simulink model "PMSM_Simulink"  (R2024b)
settings: Solver=FixedStepDiscrete  StartTime=0.0  StopTime=10  FixedStep=0.0000625/200  RelTol=1e-3
libraries: simulink x12, slpidlib x3, spsDCVoltageSourceLib x1, spsPermanentMagnetSynchronousMachineLib x1, spsUniversalBridgeLib x1, sps_lib x1
(part 1 of 2)
settings Model: SimulationMode=accelerator  PacingRate=1000  Creator=1111  LastModifiedBy=1111
settings OptimizationCC: DefaultParameterBehavior=Inlined  EnhancedBackFolding=on  PassReuseOutputArgsAs=Individual arguments  ZeroExternalMemoryAtStartup=off  ZeroInternalMemoryAtStartup=off  OptimizeBlockOrder=speed  DifferentSizesBufferReuse=on  OptimizationCustomize=off  EfficientTunableParamExpr=on
settings DebuggingCC: ParameterPrecisionLossMsg=none  ParameterTunabilityLossMsg=error
settings SFSimCC: MATLABDynamicMemAlloc=off
settings RTWCC: Description=Embedded Coder  SystemTargetFile=ert.tlc  TemplateMakefile=ert_default_tmf
settings CodeAppCC: ForceParamTrailComments=on  IgnoreCustomStorageClasses=off  OperatorAnnotations=on  SimulinkDataObjDesc=on  SFDataObjDesc=on  InsertBlockDesc=on
settings ERTTargetCC: TargetLangStandard=C99 (ISO)  GenerateSampleERTMain=on  ERTCustomFileTemplate=example_file_process.tlc

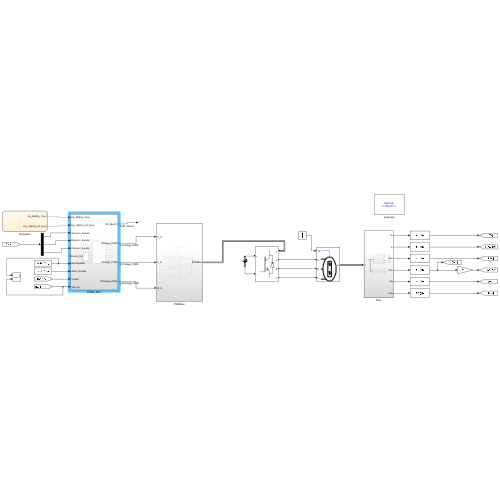
[thumbnail: Simulink's stored preview of the top-level diagram]
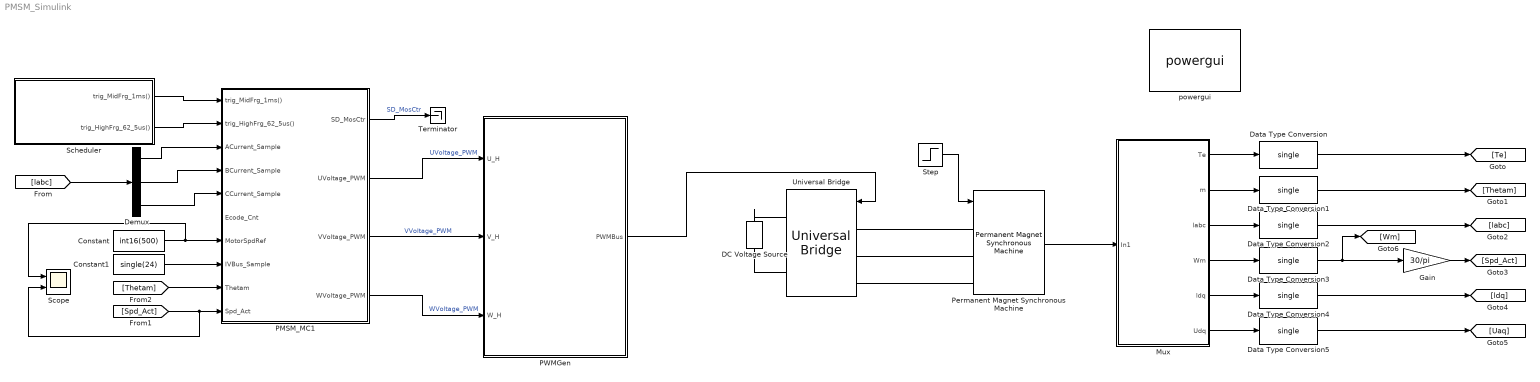
== system PMSM_Simulink ==
  Constant : Constant  Value=int16(500)  OutDataTypeStr=int16
  Constant1 : Constant  Value=single(24)
  DC Voltage Source : spsDCVoltageSourceLib/DC Voltage Source  Amplitude=24  Measurements=None
  Data Type Conversion{,1..5} (6 alike) : DataTypeConversion  OutDataTypeStr=single  SaturateOnIntegerOverflow=off  RndMeth=Floor
  Demux : Demux  Outputs=3
  Gain : Gain  Gain=30/pi
  Mux : Subsystem
  PMSM_MC1 : Subsystem
  PWMGen : Subsystem
  Permanent Magnet Synchronous Machine : spsPermanentMagnetSynchronousMachineLib/Permanent Magnet Synchronous Machine  NbPhases=3  FluxDistribution=Sinusoidal  RotorType=Salient-pole  MechanicalLoad=Torque Tm  PresetModel=No  ShowDetailedParameters=on  MeasurementBus=off  Resistance=0.51  Inductance=8.5e-3  dqInductances=[0.295e-3,0.295e-3]  La=0.00086  MachineConstant=Flux linkage established by magnets (V.s)  Flux=0.00838  VoltageCst=6.0799  TorqueCst=0.05028  Flat=120  Mechanical=[0.0000028 0 4 0 ]  PolePairs=4  InitialConditions=[0,0, 0,0]  InitialConditions5ph=[0 0 0 0 0 0]  RefAngle=Aligned with phase A axis (original Park)  IterativeDiscreteModel=Trapezoidal non iterative  TsBlock=-1  TsPowergui=0
  Scheduler : Stateflow chart  TreatAsAtomicUnit=on
  Scope : Scope  NumInputPorts=2
  Step : Step  Time=0  After=0  SampleTime=0
  Terminator : Terminator
  Universal Bridge : spsUniversalBridgeLib/Universal Bridge  Arms=3  SnubberResistance=1e5  SnubberCapacitance=inf  Device=IGBT / Diodes  Ron=1e-3  Lon=0  ForwardVoltages="[  0  0  ]"  ForwardVoltage=0  GTOparameters=[ 10e-6 , 20e-6 ]  IGBTparameters=[ 1e-6 , 2e-6 ]  Measurements=None  Measurements_2=None  converterType=Rectifier
  powergui : sps_lib/powergui  Priority=1  SimulationMode=Discrete  SampleTime=0.0000625/200  frequency=60  Iterations=50  frequencyindice=0  Pbase=100e6  ErrMax=1e-4  UnitsV=kV  UnitsW=MW  buscounter=0  FunctionMessages=off  echomessages=off  EnableUseOfTLC=off  CurrentSourceSwitches=off  DisableSnubberDevices=off  DisableRonSwitches=off  DisableVfSwitches=off  DisplayEquations=off  AutomaticDiscreteSolvers=off  SolverType=Tustin/Backward Euler (TBE)  Interpol=off  ExternalGateDelay=off  methode=off  Ts=100  x0status=blocks  SPID=on  SwTol=0  HookPort=off  NonlinearTolerance=1e-4  nMaxIteration=100  ContinueOnMaxIteration=off  RestoreLinks=warning  ResistiveCurrentMeasurement=off  Frange=[0:2:500]  Ylog=off  Xlog=on  ShowGrid=off  save=off  variable=ZData  structure=0  ZoomFFT=off  StartTime=0.0  cycles=1  DisplayStyle=1  fundamental=60  FreqAxis=off  MaxFrequency=1000  frequencyindicesteady=1  RmsSteady=1  display=off
  wires:
  Step/1 -> Permanent Magnet Synchronous Machine/1
  PWMGen/1(PWMBus) -> Universal Bridge/1
  Permanent Magnet Synchronous Machine/1 -> Mux/1(In1)
  Mux/1(Te) -> Data Type Conversion/1
  Mux/2(m) -> Data Type Conversion1/1
  Mux/3(labc) -> Data Type Conversion2/1
  Mux/4(Wm) -> Data Type Conversion3/1
  Mux/5(ldq) -> Data Type Conversion4/1
  Mux/6(Udq) -> Data Type Conversion5/1
  Data Type Conversion3/1 -> [Wm], Gain/1
  Data Type Conversion/1 -> [Te]
  Data Type Conversion1/1 -> [Thetam]
  Data Type Conversion2/1 -> [labc]
  Gain/1 -> [Spd_Act]
  Data Type Conversion4/1 -> [ldq]
  Data Type Conversion5/1 -> [Uaq]
  [labc] -> Demux/1
  PMSM_MC1/1(SD_MosCtr) -> Terminator/1  "SD_MosCtr"
  PMSM_MC1/3(VVoltage_PWM) -> PWMGen/2(V_H)  "VVoltage_PWM"
  PMSM_MC1/2(UVoltage_PWM) -> PWMGen/1(U_H)  "UVoltage_PWM"
  PMSM_MC1/4(WVoltage_PWM) -> PWMGen/3(W_H)  "WVoltage_PWM"
  Scheduler/1(trig_MidFrg_1ms()) -> PMSM_MC1/1(trig_MidFrg_1ms())
  Scheduler/2(trig_HighFrg_62_5us()) -> PMSM_MC1/2(trig_HighFrg_62_5us())
  Demux/1 -> PMSM_MC1/3(ACurrent_Sample)
  Demux/2 -> PMSM_MC1/4(BCurrent_Sample)
  Demux/3 -> PMSM_MC1/5(CCurrent_Sample)
  Constant/1 -> Scope/1, PMSM_MC1/7(MotorSpdRef)
  Constant1/1 -> PMSM_MC1/8(IVBus_Sample)
  [Thetam] -> PMSM_MC1/9(Thetam)
  [Spd_Act] -> Scope/2, PMSM_MC1/10(Spd_Act)
  connections:
  DC Voltage Source/LConn1 -- Universal Bridge/RConn2
  DC Voltage Source/RConn1 -- Universal Bridge/RConn1
  Universal Bridge/LConn2 -- Permanent Magnet Synchronous Machine/LConn2
  Universal Bridge/LConn1 -- Permanent Magnet Synchronous Machine/LConn1
  Universal Bridge/LConn3 -- Permanent Magnet Synchronous Machine/LConn3

== system PMSM_Simulink/Mux ==
  In1 : Inport
  Bus Selector : BusSelector  OutputSignals=Stator current is_a (A),Stator current is_b (A),Stator current is_c (A),Stator current is_q (A),Stator current is_d (A),Stator voltage Vs_q (V),Stator voltage Vs_d (V)
  Bus Selector1 : BusSelector  OutputSignals=Rotor speed wm (rad/s),Rotor angle thetam (rad),Electromagnetic torque Te (N*m)
  Mux : Mux  Inputs=3
  Mux1 : Mux  Inputs=2
  Mux2 : Mux  Inputs=2
  Te : Outport
  m : Outport  Port=2
  labc : Outport  Port=3
  Wm : Outport  Port=4
  ldq : Outport  Port=5
  Udq : Outport  Port=6
  wires:
  In1/1 -> Bus Selector1/1, Bus Selector/1
  Mux/1 -> labc/1
  Mux1/1 -> ldq/1
  Mux2/1 -> Udq/1
  Bus Selector/1 -> Mux/1  "<Stator current is_a (A)>"
  Bus Selector/2 -> Mux/2  "<Stator current is_b (A)>"
  Bus Selector/3 -> Mux/3  "<Stator current is_c (A)>"
  Bus Selector/4 -> Mux1/1  "<Stator current is_q (A)>"
  Bus Selector/5 -> Mux1/2  "<Stator current is_d (A)>"
  Bus Selector/6 -> Mux2/1  "<Stator voltage Vs_q (V)>"
  Bus Selector/7 -> Mux2/2  "<Stator voltage Vs_d (V)>"
  Bus Selector1/1 -> Wm/1  "<Rotor speed wm (rad/s)>"
  Bus Selector1/2 -> m/1  "<Rotor angle thetam (rad)>"
  Bus Selector1/3 -> Te/1  "<Electromagnetic torque Te (N*m)>"

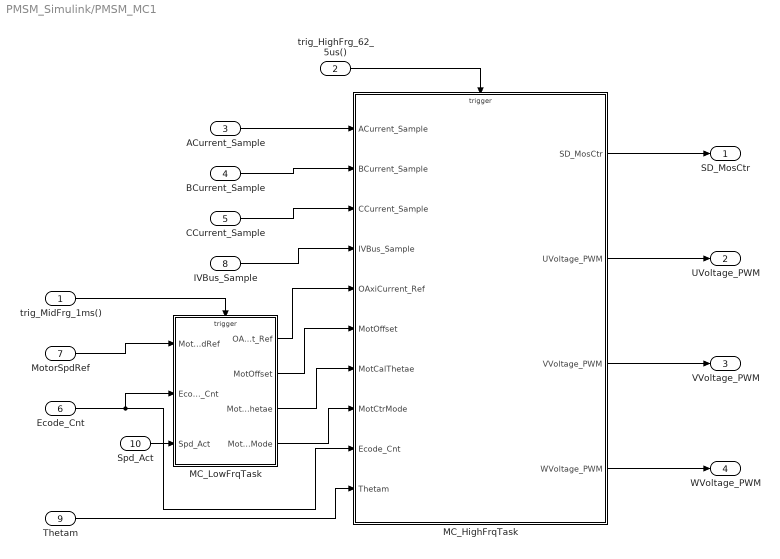
== system PMSM_Simulink/PMSM_MC1 ==
  trig_MidFrg_1ms() : Inport
  trig_HighFrg_62_5us() : Inport  Port=2
  ACurrent_Sample : Inport  Port=3
  BCurrent_Sample : Inport  Port=4
  CCurrent_Sample : Inport  Port=5
  Ecode_Cnt : Inport  Port=6
  MotorSpdRef : Inport  Port=7  OutDataTypeStr=int16
  IVBus_Sample : Inport  Port=8
  Thetam : Inport  Port=9
  Spd_Act : Inport  Port=10
  MC_HighFrqTask : Subsystem  TreatAsAtomicUnit=on
  "MC_LowFrqTask " : Subsystem  TreatAsAtomicUnit=on
  SD_MosCtr : Outport
  UVoltage_PWM : Outport  Port=2
  VVoltage_PWM : Outport  Port=3
  WVoltage_PWM : Outport  Port=4
  wires:
  trig_MidFrg_1ms()/1 -> "MC_LowFrqTask "/Trigger
  trig_HighFrg_62_5us()/1 -> MC_HighFrqTask/Trigger
  MotorSpdRef/1 -> "MC_LowFrqTask "/1(MotorSpdRef)
  Ecode_Cnt/1 -> MC_HighFrqTask/9(Ecode_Cnt), "MC_LowFrqTask "/2(Ecode_Cnt)
  ACurrent_Sample/1 -> MC_HighFrqTask/1(ACurrent_Sample)
  BCurrent_Sample/1 -> MC_HighFrqTask/2(BCurrent_Sample)
  CCurrent_Sample/1 -> MC_HighFrqTask/3(CCurrent_Sample)
  IVBus_Sample/1 -> MC_HighFrqTask/4(IVBus_Sample)
  "MC_LowFrqTask "/4(MotCtrMode) -> MC_HighFrqTask/8(MotCtrMode)
  "MC_LowFrqTask "/3(MotCalThetae) -> MC_HighFrqTask/7(MotCalThetae)
  "MC_LowFrqTask "/2(MotOffset) -> MC_HighFrqTask/6(MotOffset)
  "MC_LowFrqTask "/1(OAxiCurrent_Ref) -> MC_HighFrqTask/5(OAxiCurrent_Ref)
  MC_HighFrqTask/1(SD_MosCtr) -> SD_MosCtr/1
  MC_HighFrqTask/2(UVoltage_PWM) -> UVoltage_PWM/1
  MC_HighFrqTask/3(VVoltage_PWM) -> VVoltage_PWM/1
  MC_HighFrqTask/4(WVoltage_PWM) -> WVoltage_PWM/1
  Spd_Act/1 -> "MC_LowFrqTask "/3(Spd_Act)
  Thetam/1 -> MC_HighFrqTask/10(Thetam)

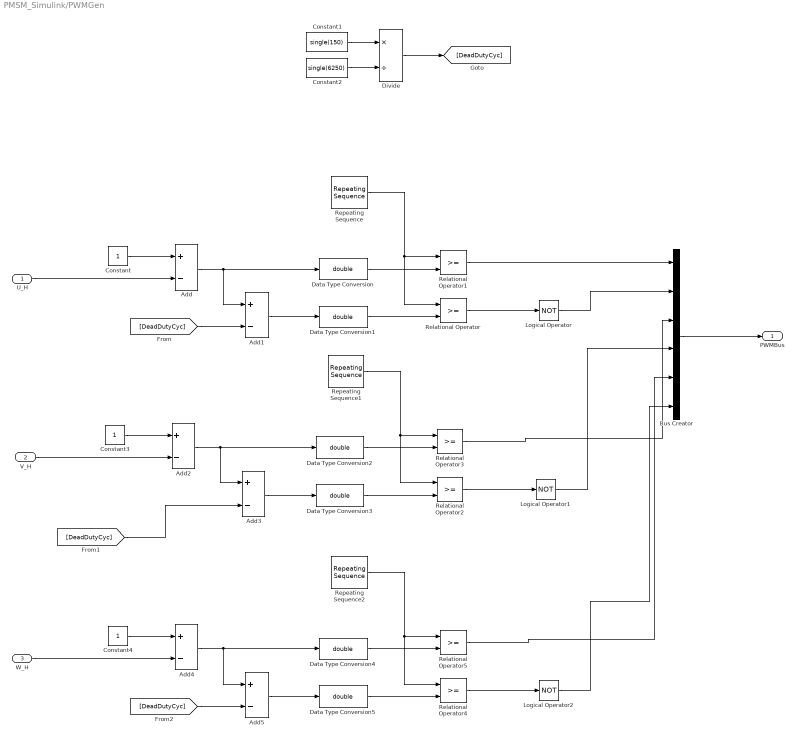
== system PMSM_Simulink/PWMGen ==
  U_H : Inport
  V_H : Inport  Port=2
  W_H : Inport  Port=3
  Add{,1..5} (6 alike) : Sum  Inputs=+-
  Bus Creator : BusCreator  Inputs=6
  Constant : Constant
  Constant1 : Constant  Value=single(150)
  Constant2 : Constant  Value=single(6250)
  Constant3 : Constant
  Constant4 : Constant
  Data Type Conversion{,1..5} (6 alike) : DataTypeConversion  OutDataTypeStr=double  SaturateOnIntegerOverflow=off  RndMeth=Floor
  Divide : Product  Inputs=*/
  Logical Operator : Logic  Operator=NOT  AllPortsSameDT=off  OutDataTypeStr=boolean
  Logical Operator1 : Logic  Operator=NOT  AllPortsSameDT=off  OutDataTypeStr=boolean
  Logical Operator2 : Logic  Operator=NOT  AllPortsSameDT=off  OutDataTypeStr=boolean
  Relational Operator{,1..5} (6 alike) : RelationalOperator  OutDataTypeStr=boolean  RndMeth=Simplest  InputSameDT=off
  Repeating Sequence : simulink/Sources/Repeating Sequence  rep_seq_t=[0 0.0000625/2 0.0000625]  rep_seq_y=[0 1 0]
  Repeating Sequence1 : simulink/Sources/Repeating Sequence  rep_seq_t=[0 0.0000625/2 0.0000625]  rep_seq_y=[0 1 0]
  Repeating Sequence2 : simulink/Sources/Repeating Sequence  rep_seq_t=[0 0.0000625/2 0.0000625]  rep_seq_y=[0 1 0]
  PWMBus : Outport
  wires:
  U_H/1 -> Add/2
  Constant/1 -> Add/1
  Add/1 -> Data Type Conversion/1, Add1/1
  Add1/1 -> Data Type Conversion1/1
  Data Type Conversion1/1 -> Relational Operator/2
  Data Type Conversion/1 -> Relational Operator1/2
  Repeating Sequence/1 -> Relational Operator/1, Relational Operator1/1
  Relational Operator/1 -> Logical Operator/1
  Relational Operator1/1 -> Bus Creator/1
  Logical Operator/1 -> Bus Creator/2
  Constant1/1 -> Divide/1
  Constant2/1 -> Divide/2
  Divide/1 -> [DeadDutyCyc]
  [DeadDutyCyc] -> Add1/2
  [DeadDutyCyc] -> Add3/2
  Relational Operator2/1 -> Logical Operator1/1
  Data Type Conversion2/1 -> Relational Operator3/2
  Data Type Conversion3/1 -> Relational Operator2/2
  Constant3/1 -> Add2/1
  Repeating Sequence1/1 -> Relational Operator2/1, Relational Operator3/1
  Add2/1 -> Data Type Conversion2/1, Add3/1
  Logical Operator1/1 -> Bus Creator/4
  V_H/1 -> Add2/2
  Add3/1 -> Data Type Conversion3/1
  Relational Operator3/1 -> Bus Creator/3
  [DeadDutyCyc] -> Add5/2
  Relational Operator4/1 -> Logical Operator2/1
  Data Type Conversion4/1 -> Relational Operator5/2
  Data Type Conversion5/1 -> Relational Operator4/2
  Constant4/1 -> Add4/1
  Repeating Sequence2/1 -> Relational Operator4/1, Relational Operator5/1
  Add4/1 -> Data Type Conversion4/1, Add5/1
  Logical Operator2/1 -> Bus Creator/6
  W_H/1 -> Add4/2
  Add5/1 -> Data Type Conversion5/1
  Relational Operator5/1 -> Bus Creator/5
  Bus Creator/1 -> PWMBus/1

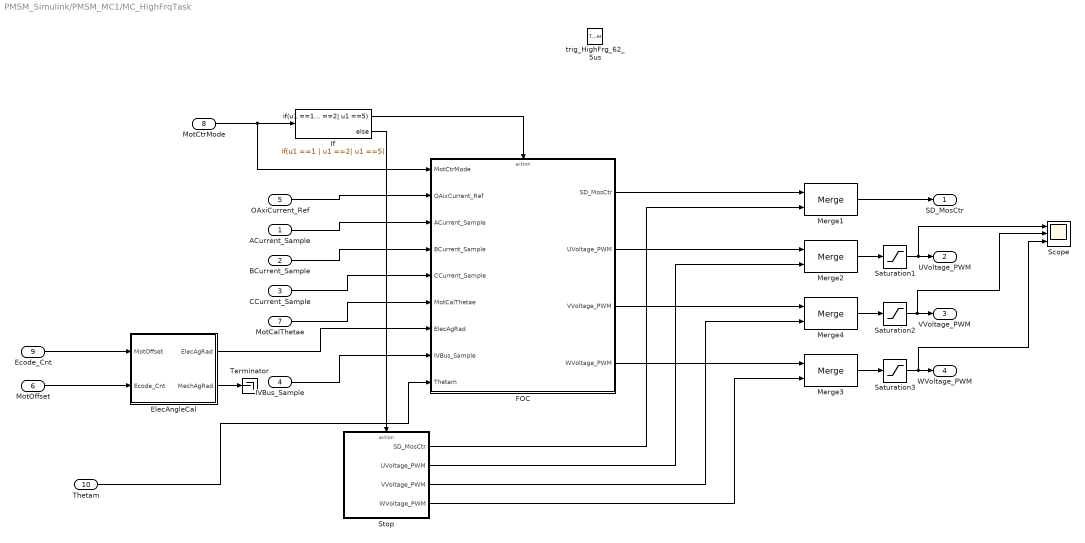
== system PMSM_Simulink/PMSM_MC1/MC_HighFrqTask ==
  ACurrent_Sample : Inport
  BCurrent_Sample : Inport  Port=2
  CCurrent_Sample : Inport  Port=3
  IVBus_Sample : Inport  Port=4
  OAxiCurrent_Ref : Inport  Port=5
  MotOffset : Inport  Port=6
  MotCalThetae : Inport  Port=7
  MotCtrMode : Inport  Port=8
  Ecode_Cnt : Inport  Port=9
  Thetam : Inport  Port=10
  trig_HighFrg_62_5us : TriggerPort  TriggerType=function-call  VariantControl=(inherit)
  ElecAngleCal : Subsystem
  FOC : Subsystem  TreatAsAtomicUnit=on
  If : If  IfExpression=u1 ==1 | u1 ==2| u1 ==5
  Merge{1..4} (4 alike) : Merge
  Saturation1 : Saturate  UpperLimit=0.95  LowerLimit=0
  Saturation2 : Saturate  UpperLimit=0.95  LowerLimit=0
  Saturation3 : Saturate  UpperLimit=0.95  LowerLimit=0
  Scope : Scope  NumInputPorts=3
  Stop : Subsystem  TreatAsAtomicUnit=on
  Terminator : Terminator
  SD_MosCtr : Outport
  UVoltage_PWM : Outport  Port=2
  VVoltage_PWM : Outport  Port=3
  WVoltage_PWM : Outport  Port=4
  wires:
  MotCtrMode/1 -> FOC/1(MotCtrMode), If/1
  If/1 -> FOC/Action
  If/2 -> Stop/Action
  FOC/1(SD_MosCtr) -> Merge1/1
  FOC/2(UVoltage_PWM) -> Merge2/1
  FOC/3(VVoltage_PWM) -> Merge4/1
  FOC/4(WVoltage_PWM) -> Merge3/1
  Stop/1(SD_MosCtr) -> Merge1/2
  Stop/2(UVoltage_PWM) -> Merge2/2
  Stop/3(VVoltage_PWM) -> Merge4/2
  Stop/4(WVoltage_PWM) -> Merge3/2
  Merge2/1 -> Saturation1/1
  Merge4/1 -> Saturation2/1
  Merge3/1 -> Saturation3/1
  Saturation1/1 -> Scope/1, UVoltage_PWM/1
  Saturation2/1 -> Scope/2, VVoltage_PWM/1
  Saturation3/1 -> Scope/3, WVoltage_PWM/1
  Merge1/1 -> SD_MosCtr/1
  Ecode_Cnt/1 -> ElecAngleCal/1(MotOffset)
  MotOffset/1 -> ElecAngleCal/2(Ecode_Cnt)
  ACurrent_Sample/1 -> FOC/3(ACurrent_Sample)
  BCurrent_Sample/1 -> FOC/4(BCurrent_Sample)
  CCurrent_Sample/1 -> FOC/5(CCurrent_Sample)
  OAxiCurrent_Ref/1 -> FOC/2(QAixCurrent_Ref)
  MotCalThetae/1 -> FOC/6(MotCalThetae)
  IVBus_Sample/1 -> FOC/8(IVBus_Sample)
  ElecAngleCal/1(ElecAgRad) -> FOC/7(ElecAgRad)
  ElecAngleCal/2(MechAgRad) -> Terminator/1
  Thetam/1 -> FOC/9(Thetam)

== system PMSM_Simulink/PMSM_MC1/MC_LowFrqTask  ==
  MotorSpdRef : Inport  OutDataTypeStr=int16
  Ecode_Cnt : Inport  Port=2
  Spd_Act : Inport  Port=3
  trig_MidFrg_1ms : TriggerPort  TriggerType=function-call  VariantControl=(inherit)
  MotModeCtr : Subsystem
  MotSpdCal : Subsystem
  SpdLoop : Subsystem
  OAxiCurrent_Ref : Outport
  MotOffset : Outport  Port=2
  MotCalThetae : Outport  Port=3
  MotCtrMode : Outport  Port=4  OutDataTypeStr=single
  wires:
  MotorSpdRef/1 -> SpdLoop/2(MotorSpdRef), MotModeCtr/2(MotorSpdRef)
  SpdLoop/1(OAxiCurrent_Ref) -> OAxiCurrent_Ref/1
  Spd_Act/1 -> SpdLoop/3(MotorActSpd)
  MotModeCtr/1(MotOffset) -> MotOffset/1
  MotModeCtr/2(MotCalThetae) -> MotCalThetae/1
  MotModeCtr/3(MotCtrMode) -> SpdLoop/1(MotorSpdRef1), MotCtrMode/1
  Ecode_Cnt/1 -> MotSpdCal/1(Ecode_Cnt), MotModeCtr/1(Ecdoe_Crt)

== system PMSM_Simulink/PMSM_MC1/MC_HighFrqTask/ElecAngleCal ==
  MotOffset : Inport
  Ecode_Cnt : Inport  Port=2
  Add : Sum  Inputs=+-
  AngleCal : Subsystem
  Demux : Demux  Outputs=2
  ElecAgRad : Outport
  MechAgRad : Outport  Port=2
  wires:
  Ecode_Cnt/1 -> Add/1
  MotOffset/1 -> Add/2
  Add/1 -> AngleCal/1(Ecode_CntCorrect)
  AngleCal/1(Theat) -> Demux/1
  Demux/2 -> ElecAgRad/1
  Demux/1 -> MechAgRad/1

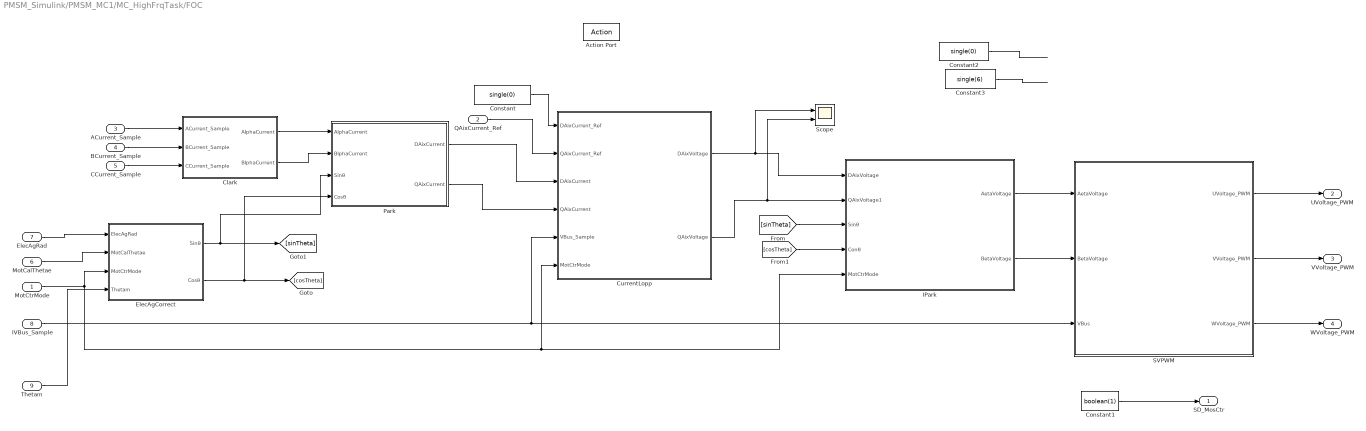
== system PMSM_Simulink/PMSM_MC1/MC_HighFrqTask/FOC ==
  MotCtrMode : Inport
  QAixCurrent_Ref : Inport  Port=2
  ACurrent_Sample : Inport  Port=3
  BCurrent_Sample : Inport  Port=4
  CCurrent_Sample : Inport  Port=5
  MotCalThetae : Inport  Port=6
  ElecAgRad : Inport  Port=7
  IVBus_Sample : Inport  Port=8
  Thetam : Inport  Port=9
  Action Port : ActionPort  ActionPortLabel=if(u1 ==1 | u1 ==2| u1 ==5)
  Clark : Subsystem
  Constant : Constant  Value=single(0)
  Constant1 : Constant  Value=boolean(1)
  Constant2 : Constant  Value=single(0)
  Constant3 : Constant  Value=single(6)
  CurrentLopp : Subsystem
  ElecAgCorrect : Subsystem
  IPark : Subsystem
  Park : Subsystem
  SVPWM : Subsystem
  Scope : Scope  NumInputPorts=2
  SD_MosCtr : Outport
  UVoltage_PWM : Outport  Port=2
  VVoltage_PWM : Outport  Port=3
  WVoltage_PWM : Outport  Port=4
  wires:
  Park/2(QAixCurrent) -> CurrentLopp/4(QAixCurrent)
  Clark/2(BIphaCurrent) -> Park/2(BIphaCurrent)
  Park/1(DAixCurrent) -> CurrentLopp/3(DAixCurrent)
  IPark/1(AetaVoltage) -> SVPWM/1(AetaVoltage)
  IPark/2(BetaVoltage) -> SVPWM/2(BetaVoltage)
  QAixCurrent_Ref/1 -> CurrentLopp/2(QAixCurrent_Ref)
  Constant/1 -> CurrentLopp/1(DAixCurrent_Ref)
  Clark/1(AIphaCurrent) -> Park/1(AIphaCurrent)
  ACurrent_Sample/1 -> Clark/1(ACurrent_Sample)
  CCurrent_Sample/1 -> Clark/3(CCurrent_Sample)
  BCurrent_Sample/1 -> Clark/2(BCurrent_Sample)
  ElecAgRad/1 -> ElecAgCorrect/1(ElecAgRad)
  MotCalThetae/1 -> ElecAgCorrect/2(MotCalThetae)
  MotCtrMode/1 -> CurrentLopp/6(MotCtrMode), IPark/5(MotCtrMode), ElecAgCorrect/3(MotCtrMode)
  ElecAgCorrect/1(Sinθ) -> Park/3(Sinθ), [sinTheta]
  ElecAgCorrect/2(Cosθ) -> Park/4(Cosθ), [cosTheta]
  [sinTheta] -> IPark/3(Sinθ)
  [cosTheta] -> IPark/4(Conθ)
  IVBus_Sample/1 -> CurrentLopp/5(VBus_Sample), SVPWM/3(VBus)
  SVPWM/2(VVoltage_PWM) -> VVoltage_PWM/1
  SVPWM/1(UVoltage_PWM) -> UVoltage_PWM/1
  SVPWM/3(WVoltage_PWM) -> WVoltage_PWM/1
  Constant1/1 -> SD_MosCtr/1
  Thetam/1 -> ElecAgCorrect/4(Thetam)
  Constant2/1 -> ?
  Constant3/1 -> ?
  CurrentLopp/2(QAixVoltage) -> Scope/2, IPark/2(QAixVoltage1)
  CurrentLopp/1(DAixVoltage) -> Scope/1, IPark/1(DAixVoltage)

== system PMSM_Simulink/PMSM_MC1/MC_HighFrqTask/Stop ==
  Action Port : ActionPort  ActionPortLabel=else
  Constant : Constant  Value=single(0)
  Constant1 : Constant  Value=boolean(0)
  SD_MosCtr : Outport
  UVoltage_PWM : Outport  Port=2
  VVoltage_PWM : Outport  Port=3
  WVoltage_PWM : Outport  Port=4
  wires:
  Constant/1 -> WVoltage_PWM/1, VVoltage_PWM/1, UVoltage_PWM/1
  Constant1/1 -> SD_MosCtr/1

== system PMSM_Simulink/PMSM_MC1/MC_LowFrqTask /MotModeCtr ==
  Ecdoe_Crt : Inport
  MotorSpdRef : Inport  Port=2  OutDataTypeStr=int16
  Chart : Stateflow chart  TreatAsAtomicUnit=on
  Compare To Constant : simulink/Logic and Bit Operations/Compare To Constant  relop=~=  const=255  OutDataTypeStr=boolean
  Constant : Constant  Value=5  OutDataTypeStr=uint8
  Switch : Switch  Criteria=u2 > Threshold  OutDataTypeStr=single  SaturateOnIntegerOverflow=off  InputSameDT=off
  MotOffset : Outport
  MotCalThetae : Outport  Port=2
  MotCtrMode : Outport  Port=3
  wires:
  Chart/2(MotOffset) -> MotOffset/1
  Chart/3(MotCalThetae) -> MotCalThetae/1
  MotorSpdRef/1 -> Chart/1(MotorSpdRef)
  Ecdoe_Crt/1 -> Chart/2(Ecode_Cnt)
  Switch/1 -> MotCtrMode/1
  Chart/1(MotCtrMode) -> Switch/3
  Compare To Constant/1 -> Switch/2
  Constant/1 -> Switch/1, Compare To Constant/1

== system PMSM_Simulink/PMSM_MC1/MC_LowFrqTask /MotSpdCal ==
  Ecode_Cnt : Inport
  Constant : Constant  Value=single(4000)
  Constant1 : Constant  Value=single(60000)
  Constant2 : Constant  Value=single(1)
  Data Type Conversion : DataTypeConversion  OutDataTypeStr=single  SaturateOnIntegerOverflow=off  RndMeth=Floor
  Delay : Delay  DelayLength=1  InitialConditionSource=Input port
      settings: InputPortMap=u0,p4
  Divide : Product  Inputs=*/
  Minus : Sum  Inputs=+-
  Product : Product
  Subsystem : Subsystem
  MotorActSpd : Outport
  wires:
  Delay/1 -> Minus/2
  Ecode_Cnt/1 -> Delay/2, Delay/1, Minus/1
  Data Type Conversion/1 -> Divide/1
  Minus/1 -> Data Type Conversion/1
  Constant/1 -> Divide/2
  Constant1/1 -> Product/2
  Divide/1 -> Product/1
  Product/1 -> Subsystem/1(In)
  Subsystem/1(MotorActSpd) -> MotorActSpd/1
  Constant2/1 -> Subsystem/2(TiCon)

== system PMSM_Simulink/PMSM_MC1/MC_LowFrqTask /SpdLoop ==
  MotorSpdRef1 : Inport
  MotorSpdRef : Inport  Port=2
  MotorActSpd : Inport  Port=3
  Compare To Constant : simulink/Logic and Bit Operations/Compare To Constant  relop===  const=5  OutDataTypeStr=boolean
  Constant1 : Constant  Value=single(6)
  Constant2 : Constant  Value=0  OutDataTypeStr=single
  Constant3 : Constant  Value=0.0001  OutDataTypeStr=single
  Constant4 : Constant  Value=0.006  OutDataTypeStr=single
  Data Type Conversion : DataTypeConversion  OutDataTypeStr=single  SaturateOnIntegerOverflow=off  RndMeth=Floor
  Discrete PID Controller : slpidlib/PID Controller  Controller=PI  Form=Parallel  TimeDomain=Discrete-time  UseExternalTs=off  SampleTime=-1  IntegratorMethod=Forward Euler  FilterMethod=Forward Euler  ControllerParametersSource=external  P=1  I=1  UseKiTs=on  D=0  UseExternalDerivativeSource=off  N=100  UseFilter=on  TunerSelectOption=Transfer Function Based (PID Tuner App)  InitialConditionSource=external  InitialConditionForIntegrator=0  InitialConditionForFilter=0  DifferentiatorICPrevScaledInput=0  ExternalReset=rising  TrackingMode=off  Kt=1  LimitOutput=off  SatLimitsSource=external  UpperSaturationLimit=inf  LowerSaturationLimit=-inf  LinearizeAsGain=off  AntiWindupMode=none  Kb=1  LimitIntegrator=on  UpperIntegratorSaturationLimit=6  LowerIntegratorSaturationLimit=-6  POutMin=[]  POutMax=[]  IOutMin=[]  IOutMax=[]  DOutMin=[]  DOutMax=[]  NOutMin=[]  NOutMax=[]  SumOutMin=[]  SumOutMax=[]  SaturationOutMin=[]  SaturationOutMax=[]  PParamMin=[]  PParamMax=[]  IParamMin=[]  IParamMax=[]  DParamMin=[]  DParamMax=[]  NParamMin=[]  NParamMax=[]  KbParamMin=[]  KbParamMax=[]  KtParamMin=[]  KtParamMax=[]  KbOutMin=[]  KbOutMax=[]  KtOutMin=[]  KtOutMax=[]  IntegratorOutMin=[]  IntegratorOutMax=[]  FilterOutMin=[]  FilterOutMax=[]  SumI1OutMin=[]  SumI1OutMax=[]  SumI2OutMin=[]  SumI2OutMax=[]  SumI3OutMin=[]  SumI3OutMax=[]  SumI4OutMin=[]  SumI4OutMax=[]  SumDOutMin=[]  SumDOutMax=[]  DifferentiatorOutMin=[]  DifferentiatorOutMax=[]  FilterDiffOutCoefMin=[]  FilterDiffOutCoefMax=[]  ReciprocalOutMin=[]  ReciprocalOutMax=[]  SumDenOutMin=[]  SumDenOutMax=[]  SumNumOutMin=[]  SumNumOutMax=[]  DivideOutMin=[]  DivideOutMax=[]  UdiffTsProdOutMin=[]  UdiffTsProdOutMax=[]  NTsProdOutMin=[]  NTsProdOutMax=[]  UintegralTsProdOutMin=[]  UintegralTsProdOutMax=[]  UngainTsProdOutMin=[]  UngainTsProdOutMax=[]  ClampingZeroOutDataTypeStr=Inherit: Inherit via back propagation  ClampingZeroOutMin=[]  ClampingZeroOutMax=[]  FilterDenConstantOutDataTypeStr=Inherit: Inherit via back propagation  FilterDenConstantOutMin=[]  FilterDenConstantOutMax=[]  PCopyOutDataTypeStr=Inherit: Inherit via back propagation  PCopyOutMin=[]  PCopyOutMax=[]  NCopyOutDataTypeStr=Inherit: Inherit via back propagation  NCopyOutMin=[]  NCopyOutMax=[]  IntegratorContinuousStateAttributes=''  IntegratorStateMustResolveToSignalObject=off  IntegratorRTWStateStorageClass=Auto  FilterContinuousStateAttributes=''  FilterStateMustResolveToSignalObject=off  FilterRTWStateStorageClass=Auto  ParallelPVariant=ExternalParameters  IdealPVariant=Disabled  IVariant=ExternalParameters  DVariant=Disabled  IntegratorVariant=Discrete  SatVariant=Disabled  AWVariant=Passthrough  PCopyVariant=Disabled  TRVariant=Disabled  FdbkBlocksVariant=Forward  IdealPFdbkVariant=Disabled  SatFdbkVariant=Disabled  DerivativeFilterVariant=Disabled  NVariant=Disabled  NCopyVariant=Disabled_SignalSpec  FilterICVariant=Disabled  IntegratorICVariant=ExternalICs  ExternalResetVariant=ExternalReset  TRSumVariant=Passthrough  SumFdbkVariant=Disabled  SumVariant=Sum_PI  TsampFilterVariant=InternalTs  TsampNgainVariant=Passthrough  TsampIntegralVariant=Disabled_SignalSpec  ExternalSaturationOutDataTypeStr=Inherit: Same as second input  DerivativeSourceVariant=Disabled  PreIntVariant=InternalPreInt
  Gain : Gain  Gain=-1
  Minus : Sum  Inputs=+-
  Saturation : Saturate  UpperLimit=5000  LowerLimit=-5000
      settings: AttributesFormatString=|
      | %<LowerLimit>
      | %<UpperLimit>
  Saturation Dynamic : simulink/Discontinuities/Saturation Dynamic  OutMin=[]  OutMax=[]  OutDataTypeStr=Inherit: Same as second input  OutDataType=fixdt(1, 16)  OutScaling=2^-10  DoSatur=off
  OAxiCurrent_Ref : Outport
  wires:
  Saturation/1 -> Data Type Conversion/1
  Data Type Conversion/1 -> Minus/1
  MotorActSpd/1 -> Minus/2
  MotorSpdRef/1 -> Saturation/1
  Constant2/1 -> Discrete PID Controller/5
  Minus/1 -> Discrete PID Controller/1
  Discrete PID Controller/1 -> Saturation Dynamic/2
  Constant1/1 -> Gain/1, Saturation Dynamic/1
  Gain/1 -> Saturation Dynamic/3
  Saturation Dynamic/1 -> OAxiCurrent_Ref/1
  Constant3/1 -> Discrete PID Controller/3
  Constant4/1 -> Discrete PID Controller/2
  Compare To Constant/1 -> Discrete PID Controller/4
  MotorSpdRef1/1 -> Compare To Constant/1

== system PMSM_Simulink/PMSM_MC1/MC_HighFrqTask/ElecAngleCal/AngleCal ==
  Ecode_CntCorrect : Inport
  If : If  IfExpression=u1 ==1  ElseIfExpressions=u1 ==-1
  If Action Subsystem1 : Subsystem  TreatAsAtomicUnit=on
  If Action Subsystem2 : Subsystem  TreatAsAtomicUnit=on
  If Action Subsystem3 : Subsystem  TreatAsAtomicUnit=on
  Merge : Merge  Inputs=3
  Sign : Signum
  Theat : Outport
  wires:
  Ecode_CntCorrect/1 -> If Action Subsystem1/1(Ecode_PhyVal), If Action Subsystem2/1(Ecode_PhyVal), Sign/1
  Sign/1 -> If/1
  If/1 -> If Action Subsystem1/Action
  If/2 -> If Action Subsystem2/Action
  If/3 -> If Action Subsystem3/Action
  If Action Subsystem2/1(Out1) -> Merge/2
  If Action Subsystem3/1(Out1) -> Merge/3
  If Action Subsystem1/1(Out1) -> Merge/1
  Merge/1 -> Theat/1

== system PMSM_Simulink/PMSM_MC1/MC_HighFrqTask/FOC/Clark ==
  ACurrent_Sample : Inport
  BCurrent_Sample : Inport  Port=2
  CCurrent_Sample : Inport  Port=3
  Gain : Gain  Gain=0.57735  OutDataTypeStr=single
  Gain1 : Gain  Gain=0.57735  OutDataTypeStr=single
  Minus : Sum  Inputs=+-
  AIphaCurrent : Outport
  BIphaCurrent : Outport  Port=2
  wires:
  Gain1/1 -> Minus/2
  BCurrent_Sample/1 -> Gain/1
  CCurrent_Sample/1 -> Gain1/1
  Minus/1 -> BIphaCurrent/1
  ACurrent_Sample/1 -> AIphaCurrent/1
  Gain/1 -> Minus/1

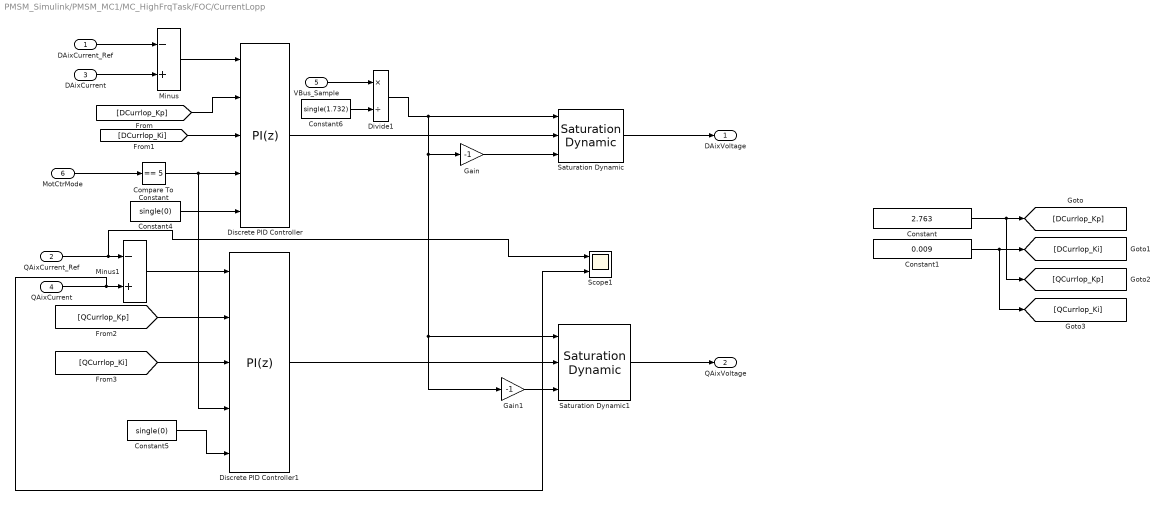
== system PMSM_Simulink/PMSM_MC1/MC_HighFrqTask/FOC/CurrentLopp ==
  DAixCurrent_Ref : Inport
  QAixCurrent_Ref : Inport  Port=2
  DAixCurrent : Inport  Port=3
  QAixCurrent : Inport  Port=4  OutDataTypeStr=single
  VBus_Sample : Inport  Port=5
  MotCtrMode : Inport  Port=6
  Compare To Constant : simulink/Logic and Bit Operations/Compare To Constant  relop===  const=5  OutDataTypeStr=boolean
  Constant : Constant  Value=2.763  OutDataTypeStr=single
  Constant1 : Constant  Value=0.009  OutDataTypeStr=single
  Constant4 : Constant  Value=single(0)
  Constant5 : Constant  Value=single(0)
  Constant6 : Constant  Value=single(1.732)
  Discrete PID Controller : slpidlib/PID Controller  Controller=PI  Form=Parallel  TimeDomain=Discrete-time  UseExternalTs=off  SampleTime=-1  IntegratorMethod=Forward Euler  FilterMethod=Forward Euler  ControllerParametersSource=external  P=1  I=1  UseKiTs=on  D=0  UseExternalDerivativeSource=off  N=100  UseFilter=on  TunerSelectOption=Transfer Function Based (PID Tuner App)  InitialConditionSource=external  InitialConditionForIntegrator=0  InitialConditionForFilter=0  DifferentiatorICPrevScaledInput=0  ExternalReset=rising  TrackingMode=off  Kt=1  LimitOutput=off  SatLimitsSource=external  UpperSaturationLimit=inf  LowerSaturationLimit=-inf  LinearizeAsGain=off  AntiWindupMode=none  Kb=1  LimitIntegrator=on  UpperIntegratorSaturationLimit=13  LowerIntegratorSaturationLimit=-13  POutMin=[]  POutMax=[]  IOutMin=[]  IOutMax=[]  DOutMin=[]  DOutMax=[]  NOutMin=[]  NOutMax=[]  SumOutMin=[]  SumOutMax=[]  SaturationOutMin=[]  SaturationOutMax=[]  PParamMin=[]  PParamMax=[]  IParamMin=[]  IParamMax=[]  DParamMin=[]  DParamMax=[]  NParamMin=[]  NParamMax=[]  KbParamMin=[]  KbParamMax=[]  KtParamMin=[]  KtParamMax=[]  KbOutMin=[]  KbOutMax=[]  KtOutMin=[]  KtOutMax=[]  IntegratorOutMin=[]  IntegratorOutMax=[]  FilterOutMin=[]  FilterOutMax=[]  SumI1OutMin=[]  SumI1OutMax=[]  SumI2OutMin=[]  SumI2OutMax=[]  SumI3OutMin=[]  SumI3OutMax=[]  SumI4OutMin=[]  SumI4OutMax=[]  SumDOutMin=[]  SumDOutMax=[]  DifferentiatorOutMin=[]  DifferentiatorOutMax=[]  FilterDiffOutCoefMin=[]  FilterDiffOutCoefMax=[]  ReciprocalOutMin=[]  ReciprocalOutMax=[]  SumDenOutMin=[]  SumDenOutMax=[]  SumNumOutMin=[]  SumNumOutMax=[]  DivideOutMin=[]  DivideOutMax=[]  UdiffTsProdOutMin=[]  UdiffTsProdOutMax=[]  NTsProdOutMin=[]  NTsProdOutMax=[]  UintegralTsProdOutMin=[]  UintegralTsProdOutMax=[]  UngainTsProdOutMin=[]  UngainTsProdOutMax=[]  ClampingZeroOutDataTypeStr=Inherit: Inherit via back propagation  ClampingZeroOutMin=[]  ClampingZeroOutMax=[]  FilterDenConstantOutDataTypeStr=Inherit: Inherit via back propagation  FilterDenConstantOutMin=[]  FilterDenConstantOutMax=[]  PCopyOutDataTypeStr=Inherit: Inherit via back propagation  PCopyOutMin=[]  PCopyOutMax=[]  NCopyOutDataTypeStr=Inherit: Inherit via back propagation  NCopyOutMin=[]  NCopyOutMax=[]  IntegratorContinuousStateAttributes=''  IntegratorStateMustResolveToSignalObject=off  IntegratorRTWStateStorageClass=Auto  FilterContinuousStateAttributes=''  FilterStateMustResolveToSignalObject=off  FilterRTWStateStorageClass=Auto  ParallelPVariant=ExternalParameters  IdealPVariant=Disabled  IVariant=ExternalParameters  DVariant=Disabled  IntegratorVariant=Discrete  SatVariant=Disabled  AWVariant=Passthrough  PCopyVariant=Disabled  TRVariant=Disabled  FdbkBlocksVariant=Forward  IdealPFdbkVariant=Disabled  SatFdbkVariant=Disabled  DerivativeFilterVariant=Disabled  NVariant=Disabled  NCopyVariant=Disabled_SignalSpec  FilterICVariant=Disabled  IntegratorICVariant=ExternalICs  ExternalResetVariant=ExternalReset  TRSumVariant=Passthrough  SumFdbkVariant=Disabled  SumVariant=Sum_PI  TsampFilterVariant=InternalTs  TsampNgainVariant=Passthrough  TsampIntegralVariant=Disabled_SignalSpec  ExternalSaturationOutDataTypeStr=Inherit: Same as second input  DerivativeSourceVariant=Disabled  PreIntVariant=InternalPreInt
  Discrete PID Controller1 : slpidlib/PID Controller  Controller=PI  Form=Parallel  TimeDomain=Discrete-time  UseExternalTs=off  SampleTime=-1  IntegratorMethod=Forward Euler  FilterMethod=Forward Euler  ControllerParametersSource=external  P=1  I=1  UseKiTs=on  D=0  UseExternalDerivativeSource=off  N=100  UseFilter=on  TunerSelectOption=Transfer Function Based (PID Tuner App)  InitialConditionSource=external  InitialConditionForIntegrator=0  InitialConditionForFilter=0  DifferentiatorICPrevScaledInput=0  ExternalReset=rising  TrackingMode=off  Kt=1  LimitOutput=off  SatLimitsSource=external  UpperSaturationLimit=inf  LowerSaturationLimit=-inf  LinearizeAsGain=off  AntiWindupMode=none  Kb=1  LimitIntegrator=on  UpperIntegratorSaturationLimit=13  LowerIntegratorSaturationLimit=-13  POutMin=[]  POutMax=[]  IOutMin=[]  IOutMax=[]  DOutMin=[]  DOutMax=[]  NOutMin=[]  NOutMax=[]  SumOutMin=[]  SumOutMax=[]  SaturationOutMin=[]  SaturationOutMax=[]  PParamMin=[]  PParamMax=[]  IParamMin=[]  IParamMax=[]  DParamMin=[]  DParamMax=[]  NParamMin=[]  NParamMax=[]  KbParamMin=[]  KbParamMax=[]  KtParamMin=[]  KtParamMax=[]  KbOutMin=[]  KbOutMax=[]  KtOutMin=[]  KtOutMax=[]  IntegratorOutMin=[]  IntegratorOutMax=[]  FilterOutMin=[]  FilterOutMax=[]  SumI1OutMin=[]  SumI1OutMax=[]  SumI2OutMin=[]  SumI2OutMax=[]  SumI3OutMin=[]  SumI3OutMax=[]  SumI4OutMin=[]  SumI4OutMax=[]  SumDOutMin=[]  SumDOutMax=[]  DifferentiatorOutMin=[]  DifferentiatorOutMax=[]  FilterDiffOutCoefMin=[]  FilterDiffOutCoefMax=[]  ReciprocalOutMin=[]  ReciprocalOutMax=[]  SumDenOutMin=[]  SumDenOutMax=[]  SumNumOutMin=[]  SumNumOutMax=[]  DivideOutMin=[]  DivideOutMax=[]  UdiffTsProdOutMin=[]  UdiffTsProdOutMax=[]  NTsProdOutMin=[]  NTsProdOutMax=[]  UintegralTsProdOutMin=[]  UintegralTsProdOutMax=[]  UngainTsProdOutMin=[]  UngainTsProdOutMax=[]  ClampingZeroOutDataTypeStr=Inherit: Inherit via back propagation  ClampingZeroOutMin=[]  ClampingZeroOutMax=[]  FilterDenConstantOutDataTypeStr=Inherit: Inherit via back propagation  FilterDenConstantOutMin=[]  FilterDenConstantOutMax=[]  PCopyOutDataTypeStr=Inherit: Inherit via back propagation  PCopyOutMin=[]  PCopyOutMax=[]  NCopyOutDataTypeStr=Inherit: Inherit via back propagation  NCopyOutMin=[]  NCopyOutMax=[]  IntegratorContinuousStateAttributes=''  IntegratorStateMustResolveToSignalObject=off  IntegratorRTWStateStorageClass=Auto  FilterContinuousStateAttributes=''  FilterStateMustResolveToSignalObject=off  FilterRTWStateStorageClass=Auto  ParallelPVariant=ExternalParameters  IdealPVariant=Disabled  IVariant=ExternalParameters  DVariant=Disabled  IntegratorVariant=Discrete  SatVariant=Disabled  AWVariant=Passthrough  PCopyVariant=Disabled  TRVariant=Disabled  FdbkBlocksVariant=Forward  IdealPFdbkVariant=Disabled  SatFdbkVariant=Disabled  DerivativeFilterVariant=Disabled  NVariant=Disabled  NCopyVariant=Disabled_SignalSpec  FilterICVariant=Disabled  IntegratorICVariant=ExternalICs  ExternalResetVariant=ExternalReset  TRSumVariant=Passthrough  SumFdbkVariant=Disabled  SumVariant=Sum_PI  TsampFilterVariant=InternalTs  TsampNgainVariant=Passthrough  TsampIntegralVariant=Disabled_SignalSpec  ExternalSaturationOutDataTypeStr=Inherit: Same as second input  DerivativeSourceVariant=Disabled  PreIntVariant=InternalPreInt
  Divide1 : Product  Inputs=*/
  Gain : Gain  Gain=-1
  Gain1 : Gain  Gain=-1
  Minus : Sum  Inputs=-+
  Minus1 : Sum  Inputs=-+
  Saturation Dynamic : simulink/Discontinuities/Saturation Dynamic  OutMin=[]  OutMax=[]  OutDataTypeStr=Inherit: Same as second input  OutDataType=fixdt(1, 16)  OutScaling=2^-10  DoSatur=off
  Saturation Dynamic1 : simulink/Discontinuities/Saturation Dynamic  OutMin=[]  OutMax=[]  OutDataTypeStr=Inherit: Same as second input  OutDataType=fixdt(1, 16)  OutScaling=2^-10  DoSatur=off
  Scope1 : Scope  NumInputPorts=3
  DAixVoltage : Outport  OutDataTypeStr=single
  QAixVoltage : Outport  Port=2  OutDataTypeStr=single
  wires:
  DAixCurrent_Ref/1 -> Minus/1
  DAixCurrent/1 -> Minus/2
  QAixCurrent_Ref/1 -> Scope1/1, Minus1/1
  QAixCurrent/1 -> Scope1/3, Minus1/2
  Minus/1 -> Discrete PID Controller/1
  Minus1/1 -> Discrete PID Controller1/1
  Constant/1 -> [QCurrlop_Kp], [DCurrlop_Kp]
  Constant1/1 -> [QCurrlop_Ki], [DCurrlop_Ki]
  [DCurrlop_Kp] -> Discrete PID Controller/2
  [DCurrlop_Ki] -> Discrete PID Controller/3
  [QCurrlop_Ki] -> Discrete PID Controller1/3
  [QCurrlop_Kp] -> Discrete PID Controller1/2
  Constant4/1 -> Discrete PID Controller/5
  Constant5/1 -> Discrete PID Controller1/5
  Discrete PID Controller/1 -> Saturation Dynamic/2
  Saturation Dynamic/1 -> DAixVoltage/1
  Saturation Dynamic1/1 -> QAixVoltage/1
  Discrete PID Controller1/1 -> Saturation Dynamic1/2
  VBus_Sample/1 -> Divide1/1
  Constant6/1 -> Divide1/2
  Divide1/1 -> Saturation Dynamic1/1, Gain1/1, Gain/1, Saturation Dynamic/1
  Gain/1 -> Saturation Dynamic/3
  Gain1/1 -> Saturation Dynamic1/3
  Compare To Constant/1 -> Discrete PID Controller1/4, Discrete PID Controller/4
  MotCtrMode/1 -> Compare To Constant/1

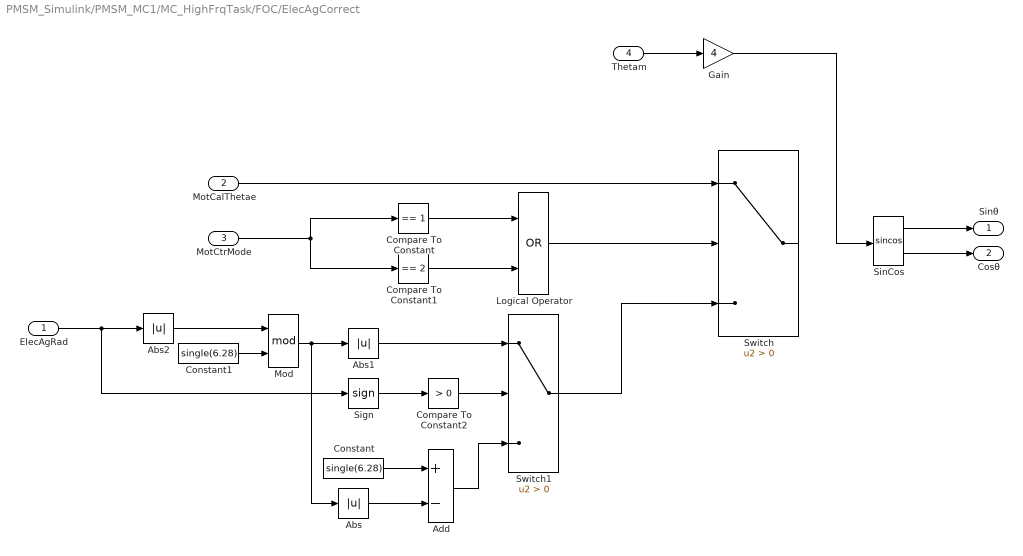
== system PMSM_Simulink/PMSM_MC1/MC_HighFrqTask/FOC/ElecAgCorrect ==
  ElecAgRad : Inport
  MotCalThetae : Inport  Port=2
  MotCtrMode : Inport  Port=3
  Thetam : Inport  Port=4
  Abs : Abs  SaturateOnIntegerOverflow=off
  Abs1 : Abs  SaturateOnIntegerOverflow=off
  Abs2 : Abs  SaturateOnIntegerOverflow=off
  Add : Sum  Inputs=+-
  Compare To Constant : simulink/Logic and Bit Operations/Compare To Constant  relop===  const=1  OutDataTypeStr=boolean
  Compare To Constant1 : simulink/Logic and Bit Operations/Compare To Constant  relop===  const=2  OutDataTypeStr=boolean
  Compare To Constant2 : simulink/Logic and Bit Operations/Compare To Constant  relop=>  const=0  OutDataTypeStr=boolean
  Constant : Constant  Value=single(6.28)
  Constant1 : Constant  Value=single(6.28)
  Gain : Gain  Gain=4
  Logical Operator : Logic  Operator=OR  AllPortsSameDT=off  OutDataTypeStr=boolean
  Mod : Math  Operator=mod
  Sign : Signum
  SinCos : Trigonometry  Operator=sincos
  Switch : Switch  Criteria=u2 > Threshold  SaturateOnIntegerOverflow=off  InputSameDT=off
  Switch1 : Switch  Criteria=u2 > Threshold  SaturateOnIntegerOverflow=off  InputSameDT=off
  Sinθ : Outport
  Cosθ : Outport  Port=2
  wires:
  MotCtrMode/1 -> Compare To Constant/1, Compare To Constant1/1
  Compare To Constant1/1 -> Logical Operator/2
  Compare To Constant/1 -> Logical Operator/1
  Logical Operator/1 -> Switch/2
  MotCalThetae/1 -> Switch/1
  Thetam/1 -> Gain/1
  SinCos/1 -> Sinθ/1
  SinCos/2 -> Cosθ/1
  Switch1/1 -> Switch/3
  Compare To Constant2/1 -> Switch1/2
  Add/1 -> Switch1/3
  Sign/1 -> Compare To Constant2/1
  Abs/1 -> Add/2
  Constant/1 -> Add/1
  Abs1/1 -> Switch1/1
  Abs2/1 -> Mod/1
  Mod/1 -> Abs/1, Abs1/1
  Constant1/1 -> Mod/2
  ElecAgRad/1 -> Sign/1, Abs2/1
  Gain/1 -> SinCos/1

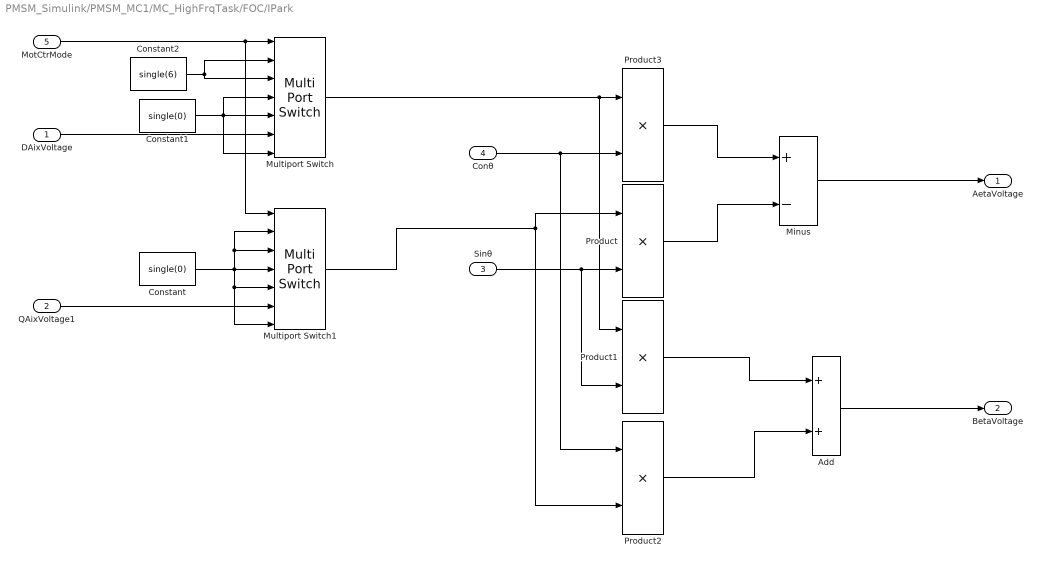
== system PMSM_Simulink/PMSM_MC1/MC_HighFrqTask/FOC/IPark ==
  DAixVoltage : Inport
  QAixVoltage1 : Inport  Port=2
  Sinθ : Inport  Port=3
  Conθ : Inport  Port=4
  MotCtrMode : Inport  Port=5
  Add : Sum  OutDataTypeStr=single
  Constant : Constant  Value=single(0)
  Constant1 : Constant  Value=single(0)
  Constant2 : Constant  Value=single(6)
  Minus : Sum  Inputs=+-  OutDataTypeStr=single
  Multiport Switch : MultiPortSwitch  Inputs=6  DiagnosticForDefault=None  SaturateOnIntegerOverflow=off  InputSameDT=off
  Multiport Switch1 : MultiPortSwitch  Inputs=6  DiagnosticForDefault=None  SaturateOnIntegerOverflow=off  InputSameDT=off
  Product{,1..3} (4 alike) : Product
  AetaVoltage : Outport
  BetaVoltage : Outport  Port=2
  wires:
  Conθ/1 -> Product2/1, Product3/2
  Sinθ/1 -> Product1/2, Product/2
  Product3/1 -> Minus/1
  Product/1 -> Minus/2
  Minus/1 -> AetaVoltage/1
  Product1/1 -> Add/1
  Product2/1 -> Add/2
  Add/1 -> BetaVoltage/1
  Multiport Switch/1 -> Product1/1, Product3/1
  Multiport Switch1/1 -> Product/1, Product2/2
  MotCtrMode/1 -> Multiport Switch1/1, Multiport Switch/1
  DAixVoltage/1 -> Multiport Switch/6
  QAixVoltage1/1 -> Multiport Switch1/6
  Constant/1 -> Multiport Switch1/7, Multiport Switch1/5, Multiport Switch1/3, Multiport Switch1/2, Multiport Switch1/4
  Constant1/1 -> Multiport Switch/7, Multiport Switch/4, Multiport Switch/5
  Constant2/1 -> Multiport Switch/3, Multiport Switch/2

== system PMSM_Simulink/PMSM_MC1/MC_HighFrqTask/FOC/Park ==
  AIphaCurrent : Inport
  BIphaCurrent : Inport  Port=2  OutDataTypeStr=single
  Sinθ : Inport  Port=3
  Cosθ : Inport  Port=4
  Add : Sum
  Add1 : Sum  Inputs=+-
  Product{,2..4} (4 alike) : Product
  DAixCurrent : Outport
  QAixCurrent : Outport  Port=2
  wires:
  AIphaCurrent/1 -> Product4/1, Product/1
  Cosθ/1 -> Product3/1, Product/2
  BIphaCurrent/1 -> Product3/2, Product2/1
  Sinθ/1 -> Product4/2, Product2/2
  Product3/1 -> Add1/1
  Product4/1 -> Add1/2
  Product/1 -> Add/1
  Product2/1 -> Add/2
  Add/1 -> DAixCurrent/1
  Add1/1 -> QAixCurrent/1

== system PMSM_Simulink/PMSM_MC1/MC_HighFrqTask/FOC/SVPWM ==
  AetaVoltage : Inport
  BetaVoltage : Inport  Port=2
  VBus : Inport  Port=3
  SevenSegSVPWM : Subsystem
  UVoltage_PWM : Outport
  VVoltage_PWM : Outport  Port=2
  WVoltage_PWM : Outport  Port=3
  wires:
  AetaVoltage/1 -> SevenSegSVPWM/1(Uα)
  BetaVoltage/1 -> SevenSegSVPWM/2(Uβ)
  VBus/1 -> SevenSegSVPWM/3(VBus)
  SevenSegSVPWM/3(WVoltage_PWM) -> WVoltage_PWM/1
  SevenSegSVPWM/1(UVoltage_PWM) -> UVoltage_PWM/1
  SevenSegSVPWM/2(VVoltage_PWM) -> VVoltage_PWM/1

== system PMSM_Simulink/PMSM_MC1/MC_LowFrqTask /MotSpdCal/Subsystem ==
  In : Inport
  TiCon : Inport  Port=2
  Add : Sum
  Add1 : Sum  Inputs=+-
  Constant : Constant
  Delay : Delay  DelayLength=1  InitialConditionSource=Input port
      settings: InputPortMap=u0,p4
  Product : Product
  Product1 : Product  OutDataTypeStr=single
  MotorActSpd : Outport
  wires:
  TiCon/1 -> Add1/2, Product/2
  Add1/1 -> Product1/1
  Constant/1 -> Add1/1
  Product/1 -> Add/1
  Product1/1 -> Add/2
  Add/1 -> Delay/1, MotorActSpd/1
  Delay/1 -> Product1/2
  In/1 -> Delay/2, Product/1

== system PMSM_Simulink/PMSM_MC1/MC_HighFrqTask/ElecAngleCal/AngleCal/If Action Subsystem1 ==
  Ecode_PhyVal : Inport
  Action Port : ActionPort  ActionPortLabel=if(u1 ==1 )
  Constant : Constant  Value=int32(4000)
  Constant1 : Constant  Value=4  OutDataTypeStr=uint8
  Constant2 : Constant  Value=single(4000)
  Constant3 : Constant  Value=single(6.28)
  Data Type Conversion : DataTypeConversion  OutDataTypeStr=single  SaturateOnIntegerOverflow=off  RndMeth=Floor
  Data Type Conversion1 : DataTypeConversion  OutDataTypeStr=single  SaturateOnIntegerOverflow=off  RndMeth=Floor
  Data Type Conversion2 : DataTypeConversion  OutDataTypeStr=single  SaturateOnIntegerOverflow=off  RndMeth=Floor
  Divide : Product  Inputs=*/
  Mod : Math  Operator=mod
  Mux : Mux  Inputs=2
  Product : Product
  Product1 : Product
  Out1 : Outport
  wires:
  Constant/1 -> Mod/2
  Ecode_PhyVal/1 -> Mod/1
  Mod/1 -> Data Type Conversion/1
  Constant3/1 -> Product/2
  Product/1 -> Mux/1, Product1/1
  Data Type Conversion1/1 -> Product1/2
  Constant1/1 -> Data Type Conversion1/1
  Product1/1 -> Data Type Conversion2/1
  Data Type Conversion2/1 -> Mux/2
  Mux/1 -> Out1/1
  Data Type Conversion/1 -> Divide/1
  Constant2/1 -> Divide/2
  Divide/1 -> Product/1

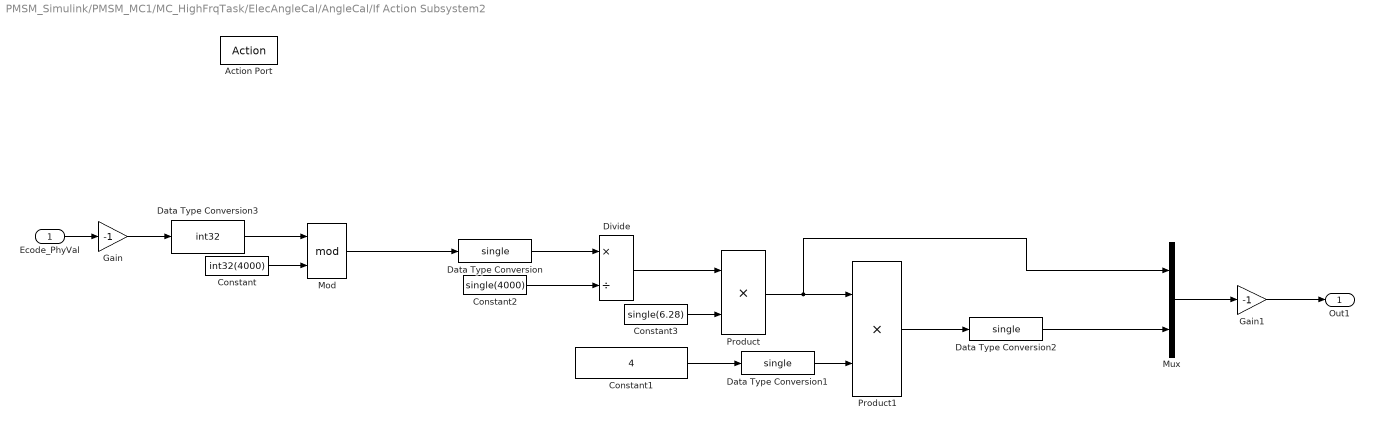
== system PMSM_Simulink/PMSM_MC1/MC_HighFrqTask/ElecAngleCal/AngleCal/If Action Subsystem2 ==
  Ecode_PhyVal : Inport
  Action Port : ActionPort  ActionPortLabel=elseif(u1 ==-1)
  Constant : Constant  Value=int32(4000)
  Constant1 : Constant  Value=4
  Constant2 : Constant  Value=single(4000)
  Constant3 : Constant  Value=single(6.28)
  Data Type Conversion : DataTypeConversion  OutDataTypeStr=single  SaturateOnIntegerOverflow=off  RndMeth=Floor
  Data Type Conversion1 : DataTypeConversion  OutDataTypeStr=single  SaturateOnIntegerOverflow=off  RndMeth=Floor
  Data Type Conversion2 : DataTypeConversion  OutDataTypeStr=single  SaturateOnIntegerOverflow=off  RndMeth=Floor
  Data Type Conversion3 : DataTypeConversion  OutDataTypeStr=int32  SaturateOnIntegerOverflow=off  RndMeth=Floor
  Divide : Product  Inputs=*/
  Gain : Gain  Gain=-1
  Gain1 : Gain  Gain=-1
  Mod : Math  Operator=mod
  Mux : Mux  Inputs=2
  Product : Product
  Product1 : Product
  Out1 : Outport
  wires:
  Data Type Conversion2/1 -> Mux/2
  Product1/1 -> Data Type Conversion2/1
  Constant1/1 -> Data Type Conversion1/1
  Mux/1 -> Gain1/1
  Data Type Conversion1/1 -> Product1/2
  Product/1 -> Mux/1, Product1/1
  Constant/1 -> Mod/2
  Ecode_PhyVal/1 -> Gain/1
  Mod/1 -> Data Type Conversion/1
  Constant3/1 -> Product/2
  Gain/1 -> Data Type Conversion3/1
  Gain1/1 -> Out1/1
  Data Type Conversion3/1 -> Mod/1
  Data Type Conversion/1 -> Divide/1
  Constant2/1 -> Divide/2
  Divide/1 -> Product/1

== system PMSM_Simulink/PMSM_MC1/MC_HighFrqTask/ElecAngleCal/AngleCal/If Action Subsystem3 ==
  Action Port : ActionPort  ActionPortLabel=else
  Constant : Constant  Value=single(0)
  Constant1 : Constant  Value=single(0)
  Mux : Mux  Inputs=2
  Out1 : Outport
  wires:
  Constant/1 -> Mux/1
  Constant1/1 -> Mux/2
  Mux/1 -> Out1/1

== system PMSM_Simulink/PMSM_MC1/MC_HighFrqTask/FOC/SVPWM/SevenSegSVPWM ==
  Uα : Inport
  Uβ : Inport  Port=2
  VBus : Inport  Port=3
  Constant : Constant  Value=single(1)
  Demux : Demux  Outputs=3
  SectorCaculate : Subsystem
  T1T2Caculate : Subsystem
  TcmCaculate : Subsystem
  XYZCaculate : Subsystem
  UVoltage_PWM : Outport
  VVoltage_PWM : Outport  Port=2
  WVoltage_PWM : Outport  Port=3
  wires:
  Uα/1 -> XYZCaculate/1(Ualpha), SectorCaculate/1(Ualpha)
  Uβ/1 -> XYZCaculate/2(Ubeta), SectorCaculate/2(Ubeta)
  SectorCaculate/1(N) -> T1T2Caculate/1(N), TcmCaculate/1(N)
  XYZCaculate/1(XYZ) -> T1T2Caculate/2(XYZ)
  T1T2Caculate/1(T1) -> TcmCaculate/2(T1)
  T1T2Caculate/2(T2) -> TcmCaculate/3(T2)
  Constant/1 -> T1T2Caculate/3(Tpwm), TcmCaculate/4(Tpwm), XYZCaculate/3(Ts)
  VBus/1 -> XYZCaculate/4(Udc)
  TcmCaculate/1(Tcm1 Tcm2 Tcm3) -> Demux/1
  Demux/3 -> WVoltage_PWM/1
  Demux/2 -> VVoltage_PWM/1
  Demux/1 -> UVoltage_PWM/1

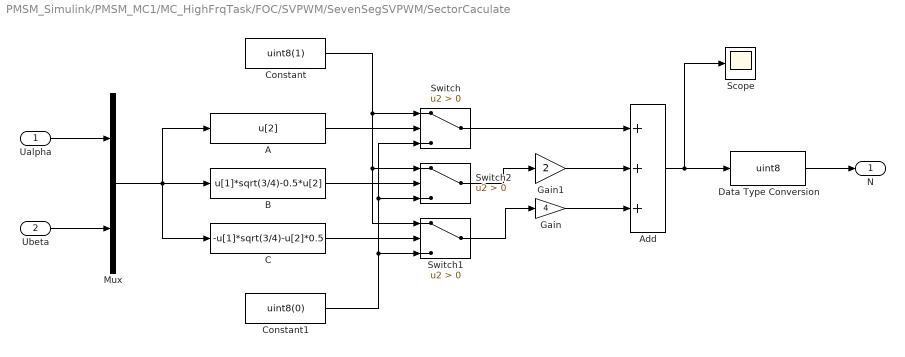
== system PMSM_Simulink/PMSM_MC1/MC_HighFrqTask/FOC/SVPWM/SevenSegSVPWM/SectorCaculate ==
  Ualpha : Inport
  Ubeta : Inport  Port=2
  A : Fcn  Expr=u[2]
  Add : Sum  Inputs=+++
  B : Fcn  Expr=u[1]*sqrt(3/4)-0.5*u[2]
  C : Fcn  Expr=-u[1]*sqrt(3/4)-u[2]*0.5
  Constant : Constant  Value=uint8(1)
  Constant1 : Constant  Value=uint8(0)
  Data Type Conversion : DataTypeConversion  OutDataTypeStr=uint8  SaturateOnIntegerOverflow=off  RndMeth=Floor
  Gain : Gain  Gain=4
  Gain1 : Gain  Gain=2
  Mux : Mux  Inputs=2
  Scope : Scope
  Switch : Switch  Criteria=u2 > Threshold  SaturateOnIntegerOverflow=off  InputSameDT=off
  Switch1 : Switch  Criteria=u2 > Threshold  SaturateOnIntegerOverflow=off  InputSameDT=off
  Switch2 : Switch  Criteria=u2 > Threshold  SaturateOnIntegerOverflow=off  InputSameDT=off
  N : Outport
  wires:
  Ualpha/1 -> Mux/1
  Ubeta/1 -> Mux/2
  Mux/1 -> C/1, A/1, B/1
  A/1 -> Switch/2
  B/1 -> Switch2/2
  C/1 -> Switch1/2
  Constant/1 -> Switch1/1, Switch2/1, Switch/1
  Constant1/1 -> Switch/3, Switch2/3, Switch1/3
  Gain/1 -> Add/3
  Gain1/1 -> Add/2
  Switch/1 -> Add/1
  Switch2/1 -> Gain1/1
  Switch1/1 -> Gain/1
  Add/1 -> Scope/1, Data Type Conversion/1
  Data Type Conversion/1 -> N/1

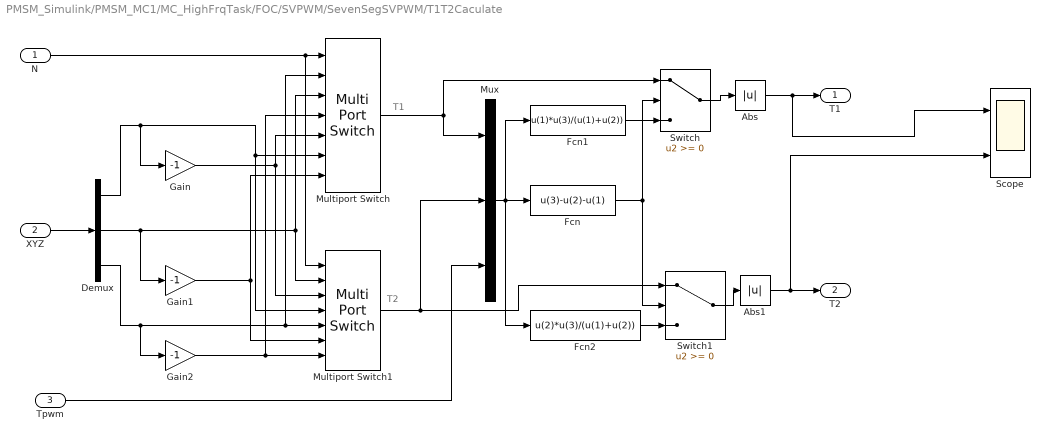
== system PMSM_Simulink/PMSM_MC1/MC_HighFrqTask/FOC/SVPWM/SevenSegSVPWM/T1T2Caculate ==
  note: T1
  note: T2
  N : Inport
  XYZ : Inport  Port=2
  Tpwm : Inport  Port=3
  Abs : Abs  SaturateOnIntegerOverflow=off
  Abs1 : Abs  SaturateOnIntegerOverflow=off
  Demux : Demux  Outputs=3
  Fcn : Fcn  Expr=u(3)-u(2)-u(1)
  Fcn1 : Fcn  Expr=u(1)*u(3)/(u(1)+u(2))
  Fcn2 : Fcn  Expr=u(2)*u(3)/(u(1)+u(2))
  Gain : Gain  Gain=-1
  Gain1 : Gain  Gain=-1
  Gain2 : Gain  Gain=-1
  Multiport Switch : MultiPortSwitch  Inputs=6  DiagnosticForDefault=None  SaturateOnIntegerOverflow=off  InputSameDT=off
  Multiport Switch1 : MultiPortSwitch  Inputs=6  DiagnosticForDefault=None  SaturateOnIntegerOverflow=off  InputSameDT=off
  Mux : Mux  Inputs=3
  Scope : Scope  NumInputPorts=2
  Switch : Switch  SaturateOnIntegerOverflow=off  InputSameDT=off
  Switch1 : Switch  SaturateOnIntegerOverflow=off  InputSameDT=off
  T1 : Outport
  T2 : Outport  Port=2
  wires:
  Gain2/1 -> Multiport Switch/4, Multiport Switch1/7
  Multiport Switch/1 -> Switch/1, Mux/1
  XYZ/1 -> Demux/1
  Gain1/1 -> Multiport Switch1/6, Multiport Switch/7
  Fcn/1 -> Switch/2, Switch1/2
  Demux/1 -> Multiport Switch/6, Multiport Switch1/4, Gain/1
  Tpwm/1 -> Mux/3
  Mux/1 -> Fcn1/1, Fcn/1, Fcn2/1
  Fcn1/1 -> Switch/3
  Demux/3 -> Multiport Switch1/5, Multiport Switch/2, Gain2/1
  Multiport Switch1/1 -> Switch1/1, Mux/2
  N/1 -> Multiport Switch/1, Multiport Switch1/1
  Fcn2/1 -> Switch1/3
  Gain/1 -> Multiport Switch1/3, Multiport Switch/5
  Demux/2 -> Multiport Switch/3, Multiport Switch1/2, Gain1/1
  Switch/1 -> Abs/1
  Switch1/1 -> Abs1/1
  Abs/1 -> Scope/1, T1/1
  Abs1/1 -> Scope/2, T2/1

== system PMSM_Simulink/PMSM_MC1/MC_HighFrqTask/FOC/SVPWM/SevenSegSVPWM/TcmCaculate ==
  N : Inport
  T1 : Inport  Port=2
  T2 : Inport  Port=3
  Tpwm : Inport  Port=4
  Fcn : Fcn  Expr=(u[3]-u[1]-u[2])/4
  Fcn1 : Fcn  Expr=(u[3]+u[1]-u[2])/4
  Fcn2 : Fcn  Expr=(u[3]+u[2]+u[1])/4
  Multiport Switch : MultiPortSwitch  Inputs=6  DiagnosticForDefault=None  SaturateOnIntegerOverflow=off  InputSameDT=off
  Multiport Switch1 : MultiPortSwitch  Inputs=6  DiagnosticForDefault=None  SaturateOnIntegerOverflow=off  InputSameDT=off
  Multiport Switch2 : MultiPortSwitch  Inputs=6  DiagnosticForDefault=None  SaturateOnIntegerOverflow=off  InputSameDT=off
  Mux : Mux  Inputs=3
  Mux1 : Mux  Inputs=3
  Tcm1 Tcm2 Tcm3 : Outport
  wires:
  Fcn/1 -> Multiport Switch/3, Multiport Switch/4, Multiport Switch1/6, Multiport Switch2/5, Multiport Switch2/7, Multiport Switch1/2
  Mux1/1 -> Tcm1 Tcm2 Tcm3/1
  Multiport Switch1/1 -> Mux1/2
  Mux/1 -> Fcn2/1, Fcn/1, Fcn1/1
  T1/1 -> Mux/1
  Fcn2/1 -> Multiport Switch/5, Multiport Switch/6, Multiport Switch1/3, Multiport Switch1/7, Multiport Switch2/2, Multiport Switch2/4
  Fcn1/1 -> Multiport Switch1/5, Multiport Switch2/3, Multiport Switch2/6, Multiport Switch1/4, Multiport Switch/7, Multiport Switch/2
  Multiport Switch2/1 -> Mux1/3
  T2/1 -> Mux/2
  N/1 -> Multiport Switch2/1, Multiport Switch1/1, Multiport Switch/1
  Multiport Switch/1 -> Mux1/1
  Tpwm/1 -> Mux/3

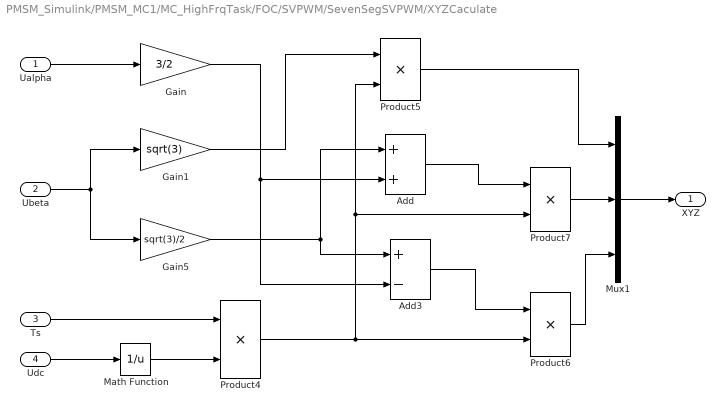
== system PMSM_Simulink/PMSM_MC1/MC_HighFrqTask/FOC/SVPWM/SevenSegSVPWM/XYZCaculate ==
  Ualpha : Inport
  Ubeta : Inport  Port=2
  Ts : Inport  Port=3
  Udc : Inport  Port=4
  Add : Sum
  Add3 : Sum  Inputs=+-
  Gain : Gain  Gain=3/2
  Gain1 : Gain  Gain=sqrt(3)
  Gain5 : Gain  Gain=sqrt(3)/2
  Math Function : Math  Operator=reciprocal  SignedPower=on
  Mux1 : Mux  Inputs=3
  Product{4..7} (4 alike) : Product  RndMeth=Zero
  XYZ : Outport
  wires:
  Product5/1 -> Mux1/1
  Math Function/1 -> Product4/2
  Mux1/1 -> XYZ/1
  Product6/1 -> Mux1/3
  Gain1/1 -> Product5/1
  Ubeta/1 -> Gain5/1, Gain1/1
  Product7/1 -> Mux1/2
  Udc/1 -> Math Function/1
  Ts/1 -> Product4/1
  Ualpha/1 -> Gain/1
  Gain5/1 -> Add/1, Add3/1
  Product4/1 -> Product6/2, Product5/2, Product7/2
  Add3/1 -> Product6/1
  Gain/1 -> Add3/2, Add/2
  Add/1 -> Product7/1

== stateflow chart PMSM_Simulink/Scheduler ==
  (default) -> (junction 7)
  (junction 7) -> (junction 9) [order 1] : [counter%%3200==3199]
  (junction 7) -> (junction 11) [order 2]
  (junction 9) -> (junction 12) : {
      | trig_MidFrg_1ms;
      | }
  (junction 12) -> (junction 11)
  (junction 11) -> (junction 33)
  (junction 33) -> (junction 41) [order 1] : [counter%%200==199]
  (junction 33) -> (junction 40) [order 2]
  (junction 41) -> (junction 34) : {
      | trig_HighFrg_62_5us;
      | }
  (junction 34) -> (junction 40)
  (junction 40) -> (junction 23)
  (junction 23) -> (junction 25) [order 1] : [counter>=1000000000]
  (junction 23) -> (junction 21) [order 2] : {
      | counter++;
      | }
  (junction 25) -> (junction 20) : {
      | counter=0;
      | }
  (junction 20) -> (junction 21)
  (junction 21) -> (junction 29)
  data: counter local int32 =0
  events: trig_MidFrg_1ms output FUNCTION_CALL_EVENT; trig_HighFrg_62_5us output FUNCTION_CALL_EVENT
